simulink model "mini_fadec"  (R2026b)
settings: Solver=VariableStepAuto  StopTime=20
PostLoadFcn:
  | run(fullfile(fileparts(get_param(bdroot, 'FileName')), 'parameters.m'));
InitFcn:
  | run(fullfile(fileparts(get_param(bdroot, 'FileName')), 'parameters.m'));
values from neighbouring files (symbols this model uses):
  c = 1.5    [parameters.m]
  dNd = %.15g;', N0, dNd))    [make_figures.m]
  k = 50    [parameters.m]
  k_true = k    (= 50)    [parameters.m]
  Ki = P.c*P.Kp/tau    [make_figures.m]
  Kp = 1/(k*tau_cl)    (= 0.04)    [parameters.m]
  Kt = 10    [parameters.m]
  m_acc = 0.20    (= 0.2)    [parameters.m]
  m_dec = 0.10    (= 0.1)    [parameters.m]
  n = 2.7    [parameters.m]
  N0 = cases{i,1}    [make_figures.m]
  rate_lim = 1    [parameters.m]
  tau_sensor = 0.02    [parameters.m]
  tau_valve = 0.08    [parameters.m]
  Ts = 0.01    [parameters.m]
  Wf0 = (N0/100)^P.n    [make_figures.m]    (also in parameters.m = (N0/100)^n; run_lin.m = (N0/100)^n)
  Wf_hi = 1.1    [parameters.m]
  Wf_lo = 0.1    [parameters.m]
libraries: simulink_extras x1, slpidlib x1, simulink x1
settings Model: Creator=a  LastModifiedBy=a

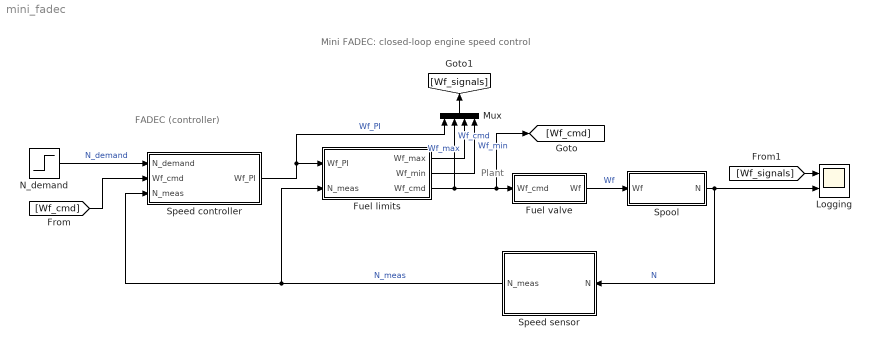
== system mini_fadec ==
  note: FADEC (controller)
  note: Mini FADEC: closed-loop engine speed control
  note: Plant
  Fuel limits : Subsystem
  Fuel valve : Subsystem
  Logging : Scope  NumInputPorts=2
      settings: ActiveDisplayYMinimum=0.01599131079675295  ActiveDisplayYMaximum=1.3462626346951421
  Mux : Mux
  N_demand : Step  Time=2  InitialValue=N0  FinalValue=N0+dNd  SampleTime=0
  Speed controller : Subsystem
  Speed sensor : Subsystem
  Spool : Subsystem
  wires:
  Spool/1(N) -> Logging/2, Speed sensor/1(N)  "N"
  Fuel valve/1(Wf) -> Spool/1(Wf)  "Wf"
  Mux/1 -> [Wf_signals]
  Speed controller/1(Wf_PI) -> Fuel limits/1(Wf_PI), Mux/1  "Wf_PI"
  N_demand/1 -> Speed controller/1(N_demand)  "N_demand"
  Fuel limits/3(Wf_cmd) -> [Wf_cmd], Fuel valve/1(Wf_cmd), Mux/2  "Wf_cmd"
  Fuel limits/1(Wf_max) -> Mux/3  "Wf_max"
  Fuel limits/2(Wf_min) -> Mux/4  "Wf_min"
  Speed sensor/1(N_meas) -> Speed controller/3(N_meas), Fuel limits/2(N_meas)  "N_meas"
  [Wf_cmd] -> Speed controller/2(Wf_cmd)
  [Wf_signals] -> Logging/1

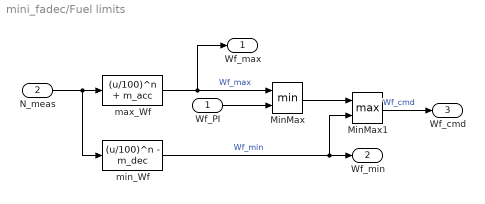
== system mini_fadec/Fuel limits ==
  Wf_PI : Inport
  N_meas : Inport  Port=2
  MinMax : MinMax  Inputs=2  ZeroCross=off
  MinMax1 : MinMax  Function=max  Inputs=2
  max_Wf : Fcn  Expr=(u/100)^n + m_acc
  min_Wf : Fcn  Expr=(u/100)^n - m_dec
  Wf_max : Outport
  Wf_min : Outport  Port=2
  Wf_cmd : Outport  Port=3
  wires:
  Wf_PI/1 -> MinMax/2
  N_meas/1 -> min_Wf/1, max_Wf/1
  max_Wf/1 -> Wf_max/1, MinMax/1  "Wf_max"
  MinMax1/1 -> Wf_cmd/1  "Wf_cmd"
  min_Wf/1 -> MinMax1/2, Wf_min/1  "Wf_min"
  MinMax/1 -> MinMax1/1

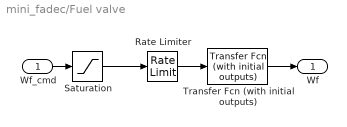
== system mini_fadec/Fuel valve ==
  Wf_cmd : Inport
  Rate Limiter : RateLimiter  RisingSlewLimit=rate_lim  SampleTimeMode=inherited  InitialCondition=Wf0
  Saturation : Saturate  UpperLimit=Wf_hi  LowerLimit=Wf_lo  ZeroCross=off
  Transfer Fcn (with initial outputs) : simulink_extras/Additional Linear/Transfer Fcn (with initial outputs)  N=[1]  D="[tau_valve  1]"  Y0=Wf0  U0=0
  Wf : Outport
  wires:
  Rate Limiter/1 -> Transfer Fcn (with initial outputs)/1
  Wf_cmd/1 -> Saturation/1
  Transfer Fcn (with initial outputs)/1 -> Wf/1
  Saturation/1 -> Rate Limiter/1

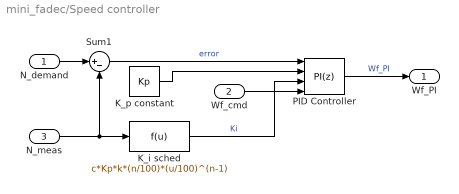
== system mini_fadec/Speed controller ==
  N_demand : Inport
  Wf_cmd : Inport  Port=2
  N_meas : Inport  Port=3
  K_i sched : Fcn  Expr=c*Kp*k*(n/100)*(u/100)^(n-1)
  K_p constant : Constant  Value=Kp
  PID Controller : slpidlib/PID Controller  Controller=PI  Form=Parallel  TimeDomain=Discrete-time  UseExternalTs=off  SampleTime=Ts  IntegratorMethod=Forward Euler  FilterMethod=Forward Euler  ControllerParametersSource=external  P=Kp  I=Ki  UseKiTs=off  D=0  UseExternalDerivativeSource=off  N=100  UseFilter=on  TunerSelectOption=Transfer Function Based (PID Tuner App)  ZeroCross=off  InitialConditionSource=internal  InitialConditionForIntegrator=Wf0  InitialConditionForFilter=Wf0  DifferentiatorICPrevScaledInput=0  ExternalReset=none  TrackingMode=on  Kt=Kt  LimitOutput=on  SatLimitsSource=internal  UpperSaturationLimit=Wf_hi  LowerSaturationLimit=Wf_lo  LinearizeAsGain=on  AntiWindupMode=none  Kb=1  LimitIntegrator=off  UpperIntegratorSaturationLimit=1.1  LowerIntegratorSaturationLimit=0.1  POutMin=[]  POutMax=[]  IOutMin=[]  IOutMax=[]  DOutMin=[]  DOutMax=[]  NOutMin=[]  NOutMax=[]  SumOutMin=[]  SumOutMax=[]  SaturationOutMin=[]  SaturationOutMax=[]  PParamMin=[]  PParamMax=[]  IParamMin=[]  IParamMax=[]  DParamMin=[]  DParamMax=[]  NParamMin=[]  NParamMax=[]  KbParamMin=[]  KbParamMax=[]  KtParamMin=[]  KtParamMax=[]  KbOutMin=[]  KbOutMax=[]  KtOutMin=[]  KtOutMax=[]  IntegratorOutMin=[]  IntegratorOutMax=[]  FilterOutMin=[]  FilterOutMax=[]  SumI1OutMin=[]  SumI1OutMax=[]  SumI2OutMin=[]  SumI2OutMax=[]  SumI3OutMin=[]  SumI3OutMax=[]  SumI4OutMin=[]  SumI4OutMax=[]  SumDOutMin=[]  SumDOutMax=[]  DifferentiatorOutMin=[]  DifferentiatorOutMax=[]  FilterDiffOutCoefMin=[]  FilterDiffOutCoefMax=[]  ReciprocalOutMin=[]  ReciprocalOutMax=[]  SumDenOutMin=[]  SumDenOutMax=[]  SumNumOutMin=[]  SumNumOutMax=[]  DivideOutMin=[]  DivideOutMax=[]  UdiffTsProdOutMin=[]  UdiffTsProdOutMax=[]  NTsProdOutMin=[]  NTsProdOutMax=[]  UintegralTsProdOutMin=[]  UintegralTsProdOutMax=[]  UngainTsProdOutMin=[]  UngainTsProdOutMax=[]  ClampingZeroOutDataTypeStr=Inherit: Inherit via back propagation  ClampingZeroOutMin=[]  ClampingZeroOutMax=[]  FilterDenConstantOutDataTypeStr=Inherit: Inherit via back propagation  FilterDenConstantOutMin=[]  FilterDenConstantOutMax=[]  PCopyOutDataTypeStr=Inherit: Inherit via back propagation  PCopyOutMin=[]  PCopyOutMax=[]  NCopyOutDataTypeStr=Inherit: Inherit via back propagation  NCopyOutMin=[]  NCopyOutMax=[]  IntegratorContinuousStateAttributes=''  IntegratorStateMustResolveToSignalObject=off  IntegratorRTWStateStorageClass=Auto  FilterContinuousStateAttributes=''  FilterStateMustResolveToSignalObject=off  FilterRTWStateStorageClass=Auto  ParallelPVariant=ExternalParameters  IdealPVariant=Disabled  IVariant=ExternalParameters  DVariant=Disabled  IntegratorVariant=Discrete  SatVariant=Enabled  AWVariant=Passthrough  PCopyVariant=Disabled  TRVariant=Enabled  FdbkBlocksVariant=Forward  IdealPFdbkVariant=Disabled  SatFdbkVariant=Disabled  DerivativeFilterVariant=Disabled  NVariant=Disabled  NCopyVariant=Disabled_SignalSpec  FilterICVariant=Disabled  IntegratorICVariant=InternalICs  ExternalResetVariant=Disabled  TRSumVariant=TrackingMode  SumFdbkVariant=Disabled  SumVariant=Sum_PI  TsampFilterVariant=InternalTs  TsampNgainVariant=Passthrough  TsampIntegralVariant=Disabled_SignalSpec  ExternalSaturationOutDataTypeStr=Inherit: Same as second input  DerivativeSourceVariant=Disabled  PreIntVariant=InternalPreInt
  Sum1 : Sum  Inputs=|+-
  Wf_PI : Outport
  wires:
  N_meas/1 -> Sum1/2, K_i sched/1
  K_p constant/1 -> PID Controller/2
  N_demand/1 -> Sum1/1
  PID Controller/1 -> Wf_PI/1  "Wf_PI"
  Wf_cmd/1 -> PID Controller/4
  K_i sched/1 -> PID Controller/3  "Ki"
  Sum1/1 -> PID Controller/1  "error"

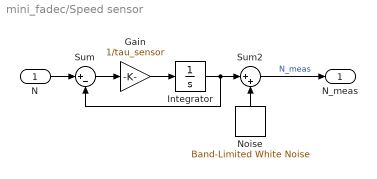
== system mini_fadec/Speed sensor ==
  N : Inport
  Gain : Gain  Gain=1/tau_sensor
  Integrator : Integrator  InitialCondition=N0
  Noise : simulink/Sources/Band-Limited White Noise  Cov=noise_power  Ts=Ts  seed=[23341]
  Sum : Sum  Inputs=|+-
  Sum2 : Sum  Inputs=|++
  N_meas : Outport
  wires:
  N/1 -> Sum/1
  Sum/1 -> Gain/1
  Sum2/1 -> N_meas/1  "N_meas"
  Noise/1 -> Sum2/2
  Integrator/1 -> Sum2/1, Sum/2
  Gain/1 -> Integrator/1

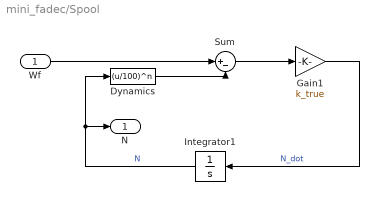
== system mini_fadec/Spool ==
  Wf : Inport
  Dynamics : Fcn  Expr=(u/100)^n
  Gain1 : Gain  Gain=k_true
  Integrator1 : Integrator  InitialCondition=N0
  Sum : Sum  Inputs=|+-
  N : Outport
  wires:
  Wf/1 -> Sum/1
  Gain1/1 -> Integrator1/1  "N_dot"
  Integrator1/1 -> Dynamics/1, N/1  "N"
  Sum/1 -> Gain1/1
  Dynamics/1 -> Sum/2
